simulink model "Prueba_kernel"  (R2025a)
settings: Solver=FixedStepDiscrete  StartTime=0.0  StopTime=1000  FixedStep=0.01  RelTol=1e-3
undefined symbols (not defined in the file or in its folder): Serial_Port, Standard_Devices
libraries: sldrtlib x1
settings Model: SimulationMode=external  Creator=aldo_  LastModifiedBy=aldo_
settings HardwareCC: ProdBitPerLong=64.0  ProdHWDeviceType=Intel->x86-64 (Linux 64)
settings RTWCC: SystemTargetFile=sldrt.tlc  TemplateMakefile=sldrt.tmf  RTWCompilerOptimization=on  Description=Simulink Desktop Real-Time
settings CodeAppCC: MaxIdLength=95.0
settings SimulinkDesktopRealTimeCC: ExtModeTransport=0.0  ExtModeStaticAllocSize=1000000.0  TargetLibSuffix=_sldrt.a  TargetPreCompLibLocation=C:\Program Files\MATLAB\R2025a\toolbox\sldrt\lib\win64  MultiwordLength=2048.0  DynamicStringBufferSize=256.0  ParMdlRefBuildCompliant=on  PreserveMATLABNamespacesInGeneratedCode=on  SubcomponentCodeInterfacePackaging=Reusable function

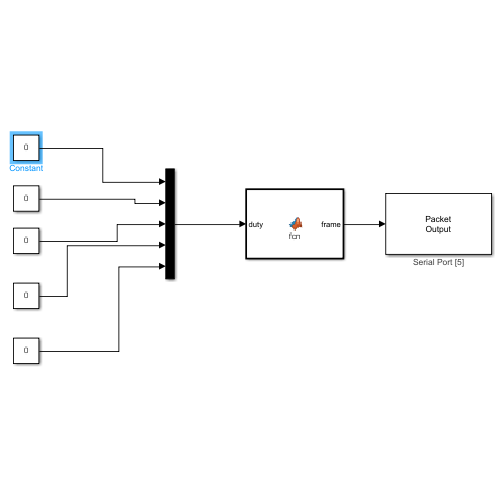
[thumbnail: Simulink's stored preview of the top-level diagram]
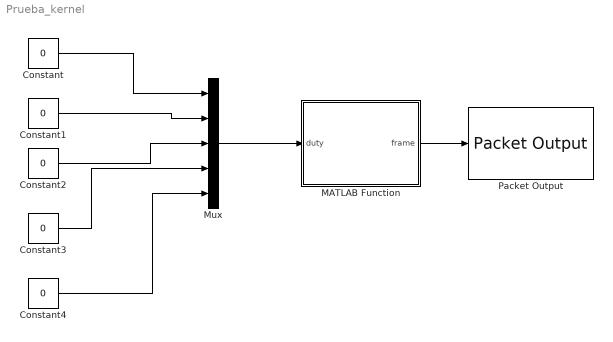
== system Prueba_kernel ==
  Constant{,1..4} (5 alike) : Constant  Value=0
  MATLAB Function : MATLAB Function  TreatAsAtomicUnit=on
  Mux : Mux  Inputs=5
  Packet Output : sldrtlib/Packet Output  SampleTime=0.01  MaxMissedTicks=10  ShowMissedTicks=off  YieldWhenWaiting=off  DrvName=Standard_Devices/Serial_Port  DrvAddress=5  DrvOptions=[115200 8 0 0 0 0 0 0]  PacketSize=14  DataTypes='14*uint8'  ShowReady=off  ShowError=off  PacketID=1  ByteOrder=1  InitialValue=[]  FinalValue=[]
      settings: AttributesFormatString=Serial Port [5]
  wires:
  Constant3/1 -> Mux/4
  Constant4/1 -> Mux/5
  Constant/1 -> Mux/1
  Constant2/1 -> Mux/3
  Constant1/1 -> Mux/2
  Mux/1 -> MATLAB Function/1(duty)
  MATLAB Function/1(frame) -> Packet Output/1

== matlab function Prueba_kernel/MATLAB Function ==
  data: duty input; frame output
function frame = fcn(duty)
  frame = armdroid_pwm_frame(duty);
